simulink model "Partie5_QPSK_Hamming"  (R2026b)
settings: Solver=FixedStepDiscrete  StopTime=Nbits*Tb
undefined symbols (not defined in the file): graine, graine_bruit, p1, Tb, variance_bruit_qpsk
libraries: simulink x2
settings Model: Creator=WORLD COMPUTERS  LastModifiedBy=WORLD COMPUTERS

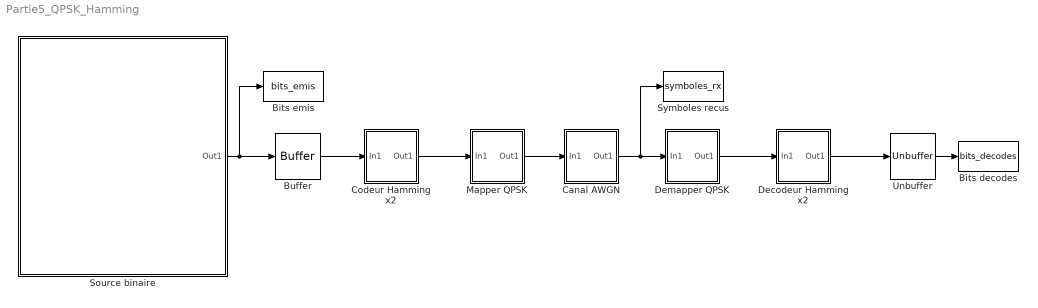
== system Partie5_QPSK_Hamming ==
  Bits decodes : ToWorkspace  VariableName=bits_decodes  SampleTime=-1
  Bits emis : ToWorkspace  VariableName=bits_emis  SampleTime=-1
  Buffer : Buffer  N=8
  Canal AWGN : Subsystem
  Codeur Hamming x2 : Subsystem
  Decodeur Hamming x2 : Subsystem
  Demapper QPSK : Subsystem
  Mapper QPSK : Subsystem
  Source binaire : Subsystem
  Symboles recus : ToWorkspace  VariableName=symboles_rx  SampleTime=-1
  Unbuffer : Unbuffer
  wires:
  Codeur Hamming x2/1(Out1) -> Mapper QPSK/1(In1)
  Source binaire/1(Out1) -> Buffer/1, Bits emis/1
  Unbuffer/1 -> Bits decodes/1
  Mapper QPSK/1(Out1) -> Canal AWGN/1(In1)
  Buffer/1 -> Codeur Hamming x2/1(In1)
  Canal AWGN/1(Out1) -> Symboles recus/1, Demapper QPSK/1(In1)
  Demapper QPSK/1(Out1) -> Decodeur Hamming x2/1(In1)
  Decodeur Hamming x2/1(Out1) -> Unbuffer/1

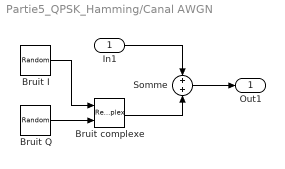
== system Partie5_QPSK_Hamming/Canal AWGN ==
  In1 : Inport
  Bruit I : RandomNumber  Variance=variance_bruit_qpsk*ones(7,1)  Seed=graine_bruit+(1:7)'  SampleTime=8*Tb
  Bruit Q : RandomNumber  Variance=variance_bruit_qpsk*ones(7,1)  Seed=graine_bruit+100+(1:7)'  SampleTime=8*Tb
  Bruit complexe : RealImagToComplex
  Somme : Sum
  Out1 : Outport
  wires:
  Bruit complexe/1 -> Somme/2
  Bruit I/1 -> Bruit complexe/1
  Bruit Q/1 -> Bruit complexe/2
  In1/1 -> Somme/1
  Somme/1 -> Out1/1

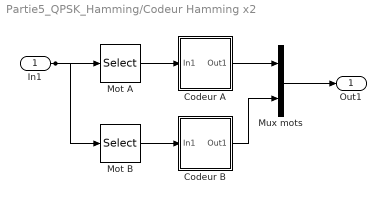
== system Partie5_QPSK_Hamming/Codeur Hamming x2 ==
  In1 : Inport
  Codeur A : Subsystem
  Codeur B : Subsystem
  Mot A : Selector  InputPortWidth=8  IndexOptions=Index vector (dialog)  Indices=[1 2 3 4]  OutputSizes=1
  Mot B : Selector  InputPortWidth=8  IndexOptions=Index vector (dialog)  Indices=[5 6 7 8]  OutputSizes=1
  Mux mots : Mux  Inputs=2
  Out1 : Outport
  wires:
  Mot B/1 -> Codeur B/1(In1)
  In1/1 -> Mot A/1, Mot B/1
  Codeur A/1(Out1) -> Mux mots/1
  Mot A/1 -> Codeur A/1(In1)
  Codeur B/1(Out1) -> Mux mots/2
  Mux mots/1 -> Out1/1

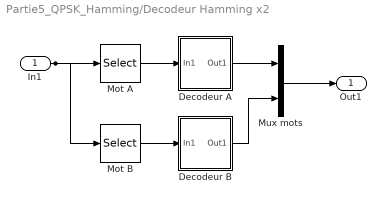
== system Partie5_QPSK_Hamming/Decodeur Hamming x2 ==
  In1 : Inport
  Decodeur A : Subsystem
  Decodeur B : Subsystem
  Mot A : Selector  InputPortWidth=14  IndexOptions=Index vector (dialog)  Indices=[1 2 3 4 5 6 7]  OutputSizes=1
  Mot B : Selector  InputPortWidth=14  IndexOptions=Index vector (dialog)  Indices=[8 9 10 11 12 13 14]  OutputSizes=1
  Mux mots : Mux  Inputs=2
  Out1 : Outport
  wires:
  Mot B/1 -> Decodeur B/1(In1)
  In1/1 -> Mot A/1, Mot B/1
  Mot A/1 -> Decodeur A/1(In1)
  Decodeur A/1(Out1) -> Mux mots/1
  Decodeur B/1(Out1) -> Mux mots/2
  Mux mots/1 -> Out1/1

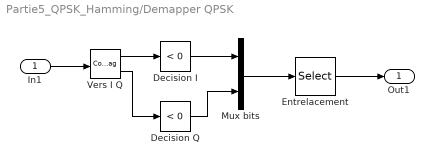
== system Partie5_QPSK_Hamming/Demapper QPSK ==
  In1 : Inport
  Decision I : simulink/Logic and Bit Operations/Compare To Constant  relop=<  const=0  OutDataTypeStr=boolean
  Decision Q : simulink/Logic and Bit Operations/Compare To Constant  relop=<  const=0  OutDataTypeStr=boolean
  Entrelacement : Selector  InputPortWidth=14  IndexOptions=Index vector (dialog)  Indices="[1   8   2   9   3  10   4  11   5  12   6  13   7  14]"  OutputSizes=1
  Mux bits : Mux  Inputs=2
  Vers I Q : ComplexToRealImag
  Out1 : Outport
  wires:
  Entrelacement/1 -> Out1/1
  In1/1 -> Vers I Q/1
  Mux bits/1 -> Entrelacement/1
  Decision Q/1 -> Mux bits/2
  Vers I Q/1 -> Decision I/1
  Vers I Q/2 -> Decision Q/1
  Decision I/1 -> Mux bits/1

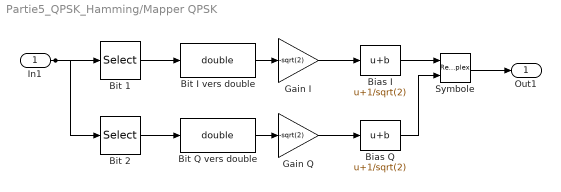
== system Partie5_QPSK_Hamming/Mapper QPSK ==
  In1 : Inport
  Bias I : Bias  Bias=1/sqrt(2)  SaturateOnIntegerOverflow=off
  Bias Q : Bias  Bias=1/sqrt(2)  SaturateOnIntegerOverflow=off
  Bit 1 : Selector  InputPortWidth=14  IndexOptions=Index vector (dialog)  Indices="[1   3   5   7   9  11  13]"  OutputSizes=1
  Bit 2 : Selector  InputPortWidth=14  IndexOptions=Index vector (dialog)  Indices="[2   4   6   8  10  12  14]"  OutputSizes=1
  Bit I vers double : DataTypeConversion  OutDataTypeStr=double  SaturateOnIntegerOverflow=off  RndMeth=Floor
  Bit Q vers double : DataTypeConversion  OutDataTypeStr=double  SaturateOnIntegerOverflow=off  RndMeth=Floor
  Gain I : Gain  Gain=-sqrt(2)
  Gain Q : Gain  Gain=-sqrt(2)
  Symbole : RealImagToComplex
  Out1 : Outport
  wires:
  In1/1 -> Bit 1/1, Bit 2/1
  Gain I/1 -> Bias I/1
  Bit I vers double/1 -> Gain I/1
  Bit Q vers double/1 -> Gain Q/1
  Bit 2/1 -> Bit Q vers double/1
  Bit 1/1 -> Bit I vers double/1
  Bias I/1 -> Symbole/1
  Gain Q/1 -> Bias Q/1
  Bias Q/1 -> Symbole/2
  Symbole/1 -> Out1/1

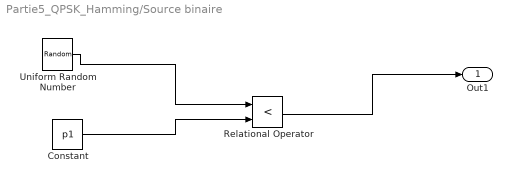
== system Partie5_QPSK_Hamming/Source binaire ==
  Constant : Constant  Value=p1
  Relational Operator : RelationalOperator  Operator=<  OutDataTypeStr=boolean  RndMeth=Simplest  InputSameDT=off
  Uniform Random Number : UniformRandomNumber  Minimum=0  Seed=graine  SampleTime=Tb
  Out1 : Outport
  wires:
  Relational Operator/1 -> Out1/1
  Constant/1 -> Relational Operator/2
  Uniform Random Number/1 -> Relational Operator/1

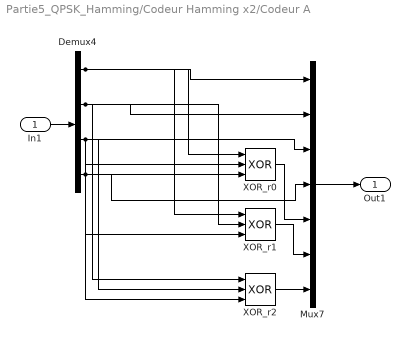
== system Partie5_QPSK_Hamming/Codeur Hamming x2/Codeur A ==
  In1 : Inport
  Demux4 : Demux
  Mux7 : Mux  Inputs=7
  XOR_r0 : Logic  Operator=XOR  Inputs=3  AllPortsSameDT=off  OutDataTypeStr=boolean
  XOR_r1 : Logic  Operator=XOR  Inputs=3  AllPortsSameDT=off  OutDataTypeStr=boolean
  XOR_r2 : Logic  Operator=XOR  Inputs=3  AllPortsSameDT=off  OutDataTypeStr=boolean
  Out1 : Outport
  wires:
  Mux7/1 -> Out1/1
  XOR_r1/1 -> Mux7/6
  XOR_r2/1 -> Mux7/7
  XOR_r0/1 -> Mux7/5
  Demux4/1 -> XOR_r1/1, XOR_r0/1, Mux7/1
  Demux4/2 -> XOR_r2/1, XOR_r1/2, Mux7/2
  Demux4/3 -> XOR_r2/2, XOR_r1/3, XOR_r0/2, Mux7/3
  Demux4/4 -> XOR_r2/3, XOR_r0/3, Mux7/4
  In1/1 -> Demux4/1

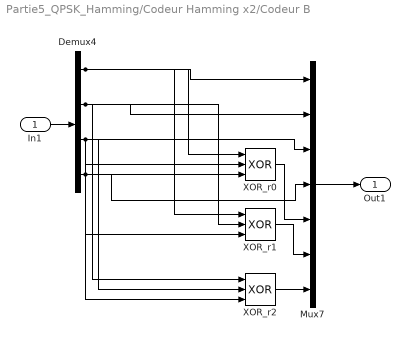
== system Partie5_QPSK_Hamming/Codeur Hamming x2/Codeur B ==
  In1 : Inport
  Demux4 : Demux
  Mux7 : Mux  Inputs=7
  XOR_r0 : Logic  Operator=XOR  Inputs=3  AllPortsSameDT=off  OutDataTypeStr=boolean
  XOR_r1 : Logic  Operator=XOR  Inputs=3  AllPortsSameDT=off  OutDataTypeStr=boolean
  XOR_r2 : Logic  Operator=XOR  Inputs=3  AllPortsSameDT=off  OutDataTypeStr=boolean
  Out1 : Outport
  wires:
  Mux7/1 -> Out1/1
  XOR_r1/1 -> Mux7/6
  XOR_r2/1 -> Mux7/7
  XOR_r0/1 -> Mux7/5
  Demux4/1 -> XOR_r1/1, XOR_r0/1, Mux7/1
  Demux4/2 -> XOR_r2/1, XOR_r1/2, Mux7/2
  Demux4/3 -> XOR_r2/2, XOR_r1/3, XOR_r0/2, Mux7/3
  Demux4/4 -> XOR_r2/3, XOR_r0/3, Mux7/4
  In1/1 -> Demux4/1

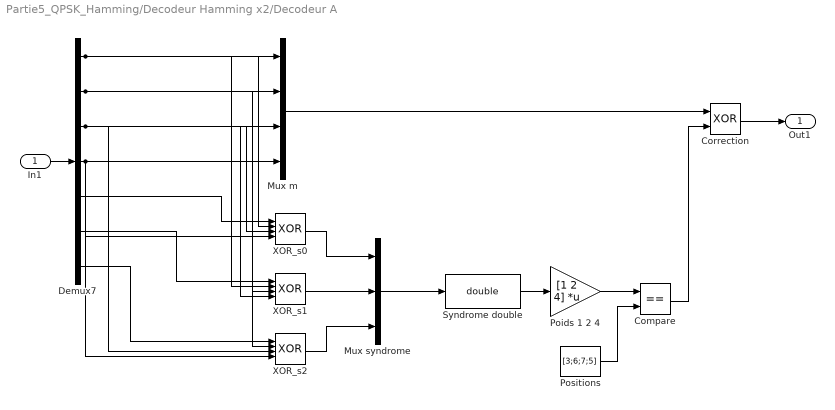
== system Partie5_QPSK_Hamming/Decodeur Hamming x2/Decodeur A ==
  In1 : Inport
  Compare : RelationalOperator  Operator===  OutDataTypeStr=boolean  RndMeth=Simplest  InputSameDT=off
  Correction : Logic  Operator=XOR  AllPortsSameDT=off  OutDataTypeStr=boolean
  Demux7 : Demux  Outputs=7
  Mux m : Mux
  Mux syndrome : Mux  Inputs=3
  Poids 1 2 4 : Gain  Gain=[1 2 4]  Multiplication=Matrix(K*u)
  Positions : Constant  Value=[3;6;7;5]
  Syndrome double : DataTypeConversion  OutDataTypeStr=double  SaturateOnIntegerOverflow=off  RndMeth=Floor
  XOR_s0 : Logic  Operator=XOR  Inputs=4  AllPortsSameDT=off  OutDataTypeStr=boolean
  XOR_s1 : Logic  Operator=XOR  Inputs=4  AllPortsSameDT=off  OutDataTypeStr=boolean
  XOR_s2 : Logic  Operator=XOR  Inputs=4  AllPortsSameDT=off  OutDataTypeStr=boolean
  Out1 : Outport
  wires:
  Correction/1 -> Out1/1
  Positions/1 -> Compare/2
  Compare/1 -> Correction/2
  Syndrome double/1 -> Poids 1 2 4/1
  Mux m/1 -> Correction/1
  Poids 1 2 4/1 -> Compare/1
  Demux7/1 -> Mux m/1, XOR_s1/2, XOR_s0/2
  XOR_s1/1 -> Mux syndrome/2
  Demux7/2 -> Mux m/2, XOR_s2/2, XOR_s1/3
  Demux7/3 -> Mux m/3, XOR_s2/3, XOR_s1/4, XOR_s0/3
  XOR_s0/1 -> Mux syndrome/1
  Demux7/4 -> Mux m/4, XOR_s2/4, XOR_s0/4
  Demux7/5 -> XOR_s0/1
  Mux syndrome/1 -> Syndrome double/1
  Demux7/6 -> XOR_s1/1
  Demux7/7 -> XOR_s2/1
  XOR_s2/1 -> Mux syndrome/3
  In1/1 -> Demux7/1

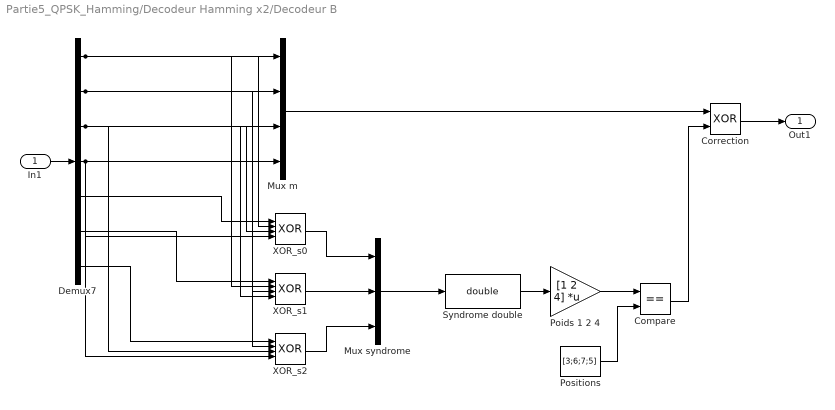
== system Partie5_QPSK_Hamming/Decodeur Hamming x2/Decodeur B ==
  In1 : Inport
  Compare : RelationalOperator  Operator===  OutDataTypeStr=boolean  RndMeth=Simplest  InputSameDT=off
  Correction : Logic  Operator=XOR  AllPortsSameDT=off  OutDataTypeStr=boolean
  Demux7 : Demux  Outputs=7
  Mux m : Mux
  Mux syndrome : Mux  Inputs=3
  Poids 1 2 4 : Gain  Gain=[1 2 4]  Multiplication=Matrix(K*u)
  Positions : Constant  Value=[3;6;7;5]
  Syndrome double : DataTypeConversion  OutDataTypeStr=double  SaturateOnIntegerOverflow=off  RndMeth=Floor
  XOR_s0 : Logic  Operator=XOR  Inputs=4  AllPortsSameDT=off  OutDataTypeStr=boolean
  XOR_s1 : Logic  Operator=XOR  Inputs=4  AllPortsSameDT=off  OutDataTypeStr=boolean
  XOR_s2 : Logic  Operator=XOR  Inputs=4  AllPortsSameDT=off  OutDataTypeStr=boolean
  Out1 : Outport
  wires:
  Correction/1 -> Out1/1
  Positions/1 -> Compare/2
  Compare/1 -> Correction/2
  Syndrome double/1 -> Poids 1 2 4/1
  Mux m/1 -> Correction/1
  Poids 1 2 4/1 -> Compare/1
  Demux7/1 -> Mux m/1, XOR_s1/2, XOR_s0/2
  XOR_s1/1 -> Mux syndrome/2
  Demux7/2 -> Mux m/2, XOR_s2/2, XOR_s1/3
  Demux7/3 -> Mux m/3, XOR_s2/3, XOR_s1/4, XOR_s0/3
  XOR_s0/1 -> Mux syndrome/1
  Demux7/4 -> Mux m/4, XOR_s2/4, XOR_s0/4
  Demux7/5 -> XOR_s0/1
  Mux syndrome/1 -> Syndrome double/1
  Demux7/6 -> XOR_s1/1
  Demux7/7 -> XOR_s2/1
  XOR_s2/1 -> Mux syndrome/3
  In1/1 -> Demux7/1
